simulink model "ARDroneSim_BatistaKF"  (R2026a)
settings: Solver=ode1  StopTime=60  FixedStep=0.005
model workspace (MAT data in the model file):
  P0 = [1  0  0  0  0  0; 0  1  0  0  0  0; 0  0  1  0  0  0; 0  0  0  0.01  0  0; 0  0  0  0  0.01  0; 0  0  0  0  0  0.01]
  Th = [0.0245  0  0; 0  0.0245  0; 0  0  0.0245]
  Xi = [0.0005894461125  0  0  0  0  0; 0  0.0005894461125  0  0  0  0; 0  0  0.0005894461125  0  0  0; 0  0  0  1e-05  0  0; 0  0  0  0  1e-05  0; 0  0  0  0  0  1e-05]
  acc_bias = [0 0 0]
  b_true_degps = [2 -3 1]
  g0 = 9.81
  seed0 = 0
  sigma_a = 0.07
  sigma_g = 0.01
  sim_A_deg = [8 6]
  sim_f_hz = [0.3 0.45]
  x0 = [0; 0; -9.81; 0; 0; 0]
settings Model: PacingRate=5

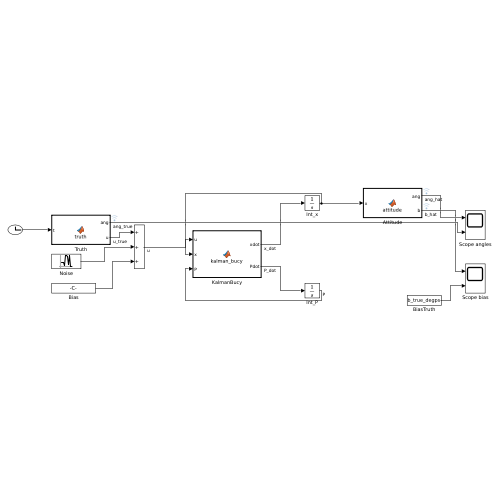
[thumbnail: Simulink's stored preview of the top-level diagram]
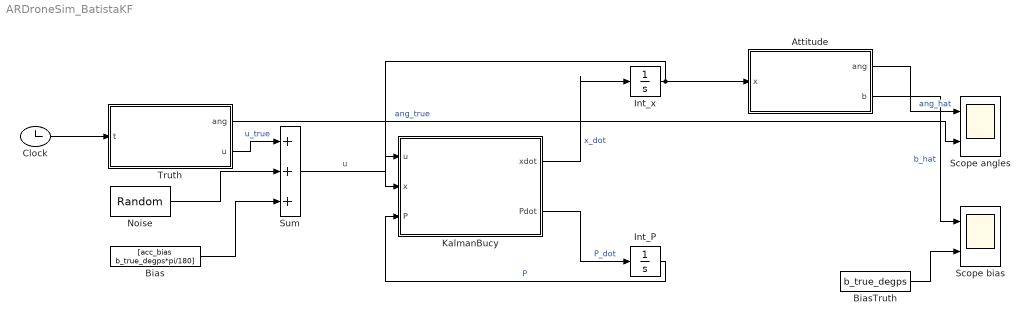
== system ARDroneSim_BatistaKF ==
  Attitude : MATLAB Function  TreatAsAtomicUnit=on
  Bias : Constant  Value=[acc_bias b_true_degps*pi/180]
  BiasTruth : Constant  Value=b_true_degps
  Clock : Clock
  Int_P : Integrator  InitialCondition=P0
  Int_x : Integrator  InitialCondition=x0
  KalmanBucy : MATLAB Function  TreatAsAtomicUnit=on
  Noise : RandomNumber  Variance=[sigma_a^2*ones(1,3) sigma_g^2*ones(1,3)]  Seed=seed0+(1:6)  SampleTime=0.005
  Scope angles : Scope  NumInputPorts=2
      settings: YLabel=Roll, pitch [deg]: KF (1) vs truth (2)
  Scope bias : Scope  NumInputPorts=2
      settings: YLabel=Gyro bias [deg/s]: KF (1) vs true (2)
  Sum : Sum  Inputs=+++
  Truth : MATLAB Function  TreatAsAtomicUnit=on
  wires:
  Clock/1 -> Truth/1(t)
  Truth/2(u) -> Sum/1  "u_true"
  Noise/1 -> Sum/2
  Bias/1 -> Sum/3
  KalmanBucy/1(xdot) -> Int_x/1  "x_dot"
  KalmanBucy/2(Pdot) -> Int_P/1  "P_dot"
  Int_x/1 -> KalmanBucy/2(x), Attitude/1(x)
  Int_P/1 -> KalmanBucy/3(P)  "P"
  Sum/1 -> KalmanBucy/1(u)  "u"
  Attitude/1(ang) -> Scope angles/1  "ang_hat"
  Truth/1(ang) -> Scope angles/2  "ang_true"
  Attitude/2(b) -> Scope bias/1  "b_hat"
  BiasTruth/1 -> Scope bias/2

== matlab function ARDroneSim_BatistaKF/KalmanBucy ==
  data: u input; xdot output; x input; P input; Pdot output; Xi parameter; Th parameter
function [xdot, Pdot] = kalman_bucy(u, x, P, Xi, Th)
% Continuous-time Kalman filter for the Batista et al. system (2)/(10).
% u = [accelerometer (m/s^2); rate gyro (rad/s)], x = [x1; bias], P: 6x6.
y = u(1:3);  w = u(4:6);
Sw = [0 -w(3) w(2); w(3) 0 -w(1); -w(2) w(1) 0];
Sy = [0 -y(3) y(2); y(3) 0 -y(1); -y(2) y(1) 0];
A  = [-Sw -Sy; zeros(3) zeros(3)];
C  = [eye(3) zeros(3)];
K  = P*C' / Th;
xdot = A*x + K*(y - C*x);
Pdot = A*P + P*A' + Xi - K*(C*P);
end

== matlab function ARDroneSim_BatistaKF/Truth ==
  data: t input; ang output; u output; sim_A_deg parameter; sim_f_hz parameter; g0 parameter
function [ang, u] = truth(t, sim_A_deg, sim_f_hz, g0)
% Exact [roll; pitch] [deg] and u = [accelerometer (m/s^2); rate gyro (rad/s)].
A = sim_A_deg*pi/180;  f = sim_f_hz;
ph = A(1)*sin(2*pi*f(1)*t);              dph = A(1)*2*pi*f(1)*cos(2*pi*f(1)*t);
th = A(2)*sin(2*pi*f(2)*t + pi/3);       dth = A(2)*2*pi*f(2)*cos(2*pi*f(2)*t + pi/3);
w = [dph; dth*cos(ph); -dth*sin(ph)];
y = g0*[sin(th); -sin(ph)*cos(th); -cos(ph)*cos(th)];
ang = [ph; th]*180/pi;
u = [y; w];
end

== matlab function ARDroneSim_BatistaKF/Attitude ==
  data: x input; ang output; b output
function [ang, b] = attitude(x)
% Roll/pitch [deg] from the filtered body-frame vector (sensor convention
% az = -g at rest) and gyro bias estimate [deg/s].
x1 = x(1:3);
n  = norm(x1);
phi = atan2(-x1(2), -x1(3))*180/pi;
if n > eps
    theta = asin(x1(1)/n)*180/pi;
else
    theta = 0;
end
ang = [phi; theta];
b = x(4:6)*180/pi;
end
